simulink model "Completo"  (R2026b)
settings: Solver=ode45  StopTime=10  MaxStep=0.005
libraries: simulink_extras x5
settings Model: Creator=Usuario  LastModifiedBy=Usuario
settings DebuggingCC: UnderSpecifiedDimensionMsg=warning

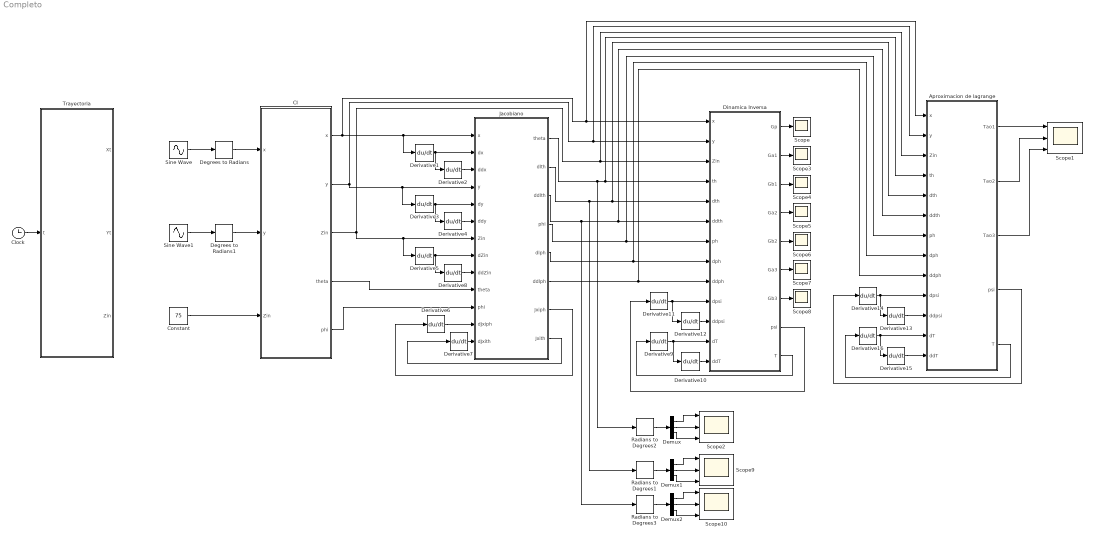
== system Completo ==
  Aproximacion de lagrange : MATLAB Function  TreatAsAtomicUnit=on
  CI : MATLAB Function  TreatAsAtomicUnit=on
  Clock : Clock
  Constant : Constant  Value=75
  Degrees to Radians : simulink_extras/Transformations/Degrees to Radians
  Degrees to Radians1 : simulink_extras/Transformations/Degrees to Radians
  Demux : Demux  Outputs=3
  Demux1 : Demux  Outputs=3
  Demux2 : Demux  Outputs=3
  Derivative{1..16} (16 alike) : Derivative
  Dinamica Inversa : MATLAB Function  TreatAsAtomicUnit=on
  Jacobiano : MATLAB Function  TreatAsAtomicUnit=on
  Radians to Degrees1 : simulink_extras/Transformations/Radians to Degrees
  Radians to Degrees2 : simulink_extras/Transformations/Radians to Degrees
  Radians to Degrees3 : simulink_extras/Transformations/Radians to Degrees
  Scope{,3..8} (7 alike) : Scope
      Scope settings: ActiveDisplayYMinimum=-37.545349688525228  ActiveDisplayYMaximum=37.17658468339345
      Scope3 settings: ActiveDisplayYMinimum=-18.564193111964496  ActiveDisplayYMaximum=37.368196271404251  DataLoggingVariableName=ScopeData3
      Scope4 settings: ActiveDisplayYMinimum=-1  ActiveDisplayYMaximum=1  DataLoggingVariableName=ScopeData4
      Scope5 settings: ActiveDisplayYMinimum=-21.313116337921368  ActiveDisplayYMaximum=32.9435376296142  DataLoggingVariableName=ScopeData5
      Scope6 settings: ActiveDisplayYMinimum=-1  ActiveDisplayYMaximum=1  DataLoggingVariableName=ScopeData6
      Scope7 settings: ActiveDisplayYMinimum=-1  ActiveDisplayYMaximum=1  DataLoggingVariableName=ScopeData7
      Scope8 settings: ActiveDisplayYMinimum=-1  ActiveDisplayYMaximum=1  DataLoggingVariableName=ScopeData8
  Scope{1..2,9..10} (4 alike) : Scope  NumInputPorts=3
      Scope1 settings: ActiveDisplayYMinimum=-0.0048170344652643951  ActiveDisplayYMaximum=-0.0041912233982996754
      Scope10 settings: ActiveDisplayYMinimum=-5322.94377337578  ActiveDisplayYMaximum=5538.32074002052  DataLoggingVariableName=ScopeData10
      Scope2 settings: ActiveDisplayYMinimum=-267.38871393580234  ActiveDisplayYMaximum=-108.53520217148704  DataLoggingVariableName=ScopeData2
      Scope9 settings: ActiveDisplayYMinimum=-34.793520974739913  ActiveDisplayYMaximum=34.948790472185514  DataLoggingVariableName=ScopeData9
  Sine Wave : Sin  Amplitude=10  Frequency=0.5*pi  SampleTime=0
  Sine Wave1 : Sin  Amplitude=10  Frequency=0.5*pi  Phase=pi/2  SampleTime=0
  Trayectoria : MATLAB Function  TreatAsAtomicUnit=on
  wires:
  Derivative6/1 -> Jacobiano/12(dJxiph)
  Derivative7/1 -> Jacobiano/13(dJxith)
  Derivative2/1 -> Jacobiano/3(ddx)
  Derivative1/1 -> Derivative2/1, Jacobiano/2(dx)
  Derivative3/1 -> Jacobiano/5(dy), Derivative4/1
  Derivative4/1 -> Jacobiano/6(ddy)
  Derivative5/1 -> Jacobiano/8(dZin), Derivative8/1
  Derivative8/1 -> Jacobiano/9(ddZin)
  CI/4(theta) -> Jacobiano/10("theta ")
  CI/5(phi) -> Jacobiano/11("phi ")
  Jacobiano/8(Jxith) -> Derivative7/1
  Jacobiano/7(Jxiph) -> Derivative6/1
  Dinamica Inversa/3(Gb1) -> Scope4/1
  Dinamica Inversa/1(Gp) -> Scope/1
  Dinamica Inversa/2(Ga1) -> Scope3/1
  Dinamica Inversa/7(Gb3) -> Scope8/1
  Dinamica Inversa/6(Ga3) -> Scope7/1
  Dinamica Inversa/4(Ga2) -> Scope5/1
  CI/2(y) -> Jacobiano/4(y), Derivative3/1, Dinamica Inversa/2(y), Aproximacion de lagrange/2(y)
  CI/1(x) -> Aproximacion de lagrange/1(x), Dinamica Inversa/1(x), Jacobiano/1(x), Derivative1/1
  Derivative10/1 -> Dinamica Inversa/13(ddT)
  Derivative12/1 -> Dinamica Inversa/11(ddpsi)
  Dinamica Inversa/8(psi) -> Derivative11/1
  Jacobiano/5(dlph) -> Aproximacion de lagrange/8(dph), Dinamica Inversa/8(dph)
  Dinamica Inversa/5(Gb2) -> Scope6/1
  Jacobiano/1(theta) -> Radians to Degrees2/1, Aproximacion de lagrange/4(th), Dinamica Inversa/4(th)
  Jacobiano/6(ddlph) -> Aproximacion de lagrange/9(ddph), Dinamica Inversa/9(ddph)
  Jacobiano/4(phi) -> Aproximacion de lagrange/7(ph), Dinamica Inversa/7(ph)
  Derivative9/1 -> Dinamica Inversa/12(dT), Derivative10/1
  Dinamica Inversa/9(T) -> Derivative9/1
  Derivative11/1 -> Derivative12/1, Dinamica Inversa/10(dpsi)
  Jacobiano/2(dlth) -> Radians to Degrees1/1, Aproximacion de lagrange/5(dth), Dinamica Inversa/5(dth)
  CI/3(Zin) -> Derivative5/1, Jacobiano/7(Zin), Aproximacion de lagrange/3(Zin), Dinamica Inversa/3(Zin)
  Derivative13/1 -> Aproximacion de lagrange/11(ddpsi)
  Derivative14/1 -> Derivative13/1, Aproximacion de lagrange/10(dpsi)
  Derivative15/1 -> Aproximacion de lagrange/13(ddT)
  Derivative16/1 -> Derivative15/1, Aproximacion de lagrange/12(dT)
  Aproximacion de lagrange/5(T) -> Derivative16/1
  Aproximacion de lagrange/4(psi) -> Derivative14/1
  Aproximacion de lagrange/1(Tao1) -> Scope1/1
  Aproximacion de lagrange/2(Tao2) -> Scope1/2
  Aproximacion de lagrange/3(Tao3) -> Scope1/3
  Clock/1 -> Trayectoria/1(t)
  Demux/3 -> Scope2/3
  Demux/1 -> Scope2/1
  Demux/2 -> Scope2/2
  Radians to Degrees2/1 -> Demux/1
  Radians to Degrees1/1 -> Demux1/1
  Demux1/2 -> Scope9/2
  Demux1/1 -> Scope9/1
  Demux1/3 -> Scope9/3
  Demux2/3 -> Scope10/3
  Demux2/1 -> Scope10/1
  Demux2/2 -> Scope10/2
  Radians to Degrees3/1 -> Demux2/1
  Jacobiano/3(ddlth) -> Radians to Degrees3/1, Aproximacion de lagrange/6(ddth), Dinamica Inversa/6(ddth)
  Constant/1 -> CI/3("Zin ")
  Sine Wave/1 -> Degrees to Radians/1
  Degrees to Radians/1 -> CI/1("x ")
  Sine Wave1/1 -> Degrees to Radians1/1
  Degrees to Radians1/1 -> CI/2("y ")

== matlab function Completo/Dinamica Inversa ==
  data: Gp output size=[9,1]; Ga1 output size=[9,1]; Gb1 output size=[9,1]; x input size=[1,1]; Ga2 output size=[9,1]; y input size=[1,1]; Zin input size=[1,1]; Gb2 output size=[9,1]; th input size=[3,1]; dth input size=[3,1]; ddth input size=[3,1]; ph input size=[3,1]; dph input size=[3,1]; ddph input size=[3,1]; dpsi input size=[3,1]; ddpsi input size=[3,1]; dT input size=[3,1]; ddT input size=[3,1]; Ga3 output size=[9,1]; Gb3 output size=[9,1]; psi output size=[3,1]; T output size=[3,1]
function [Gp, Ga1, Gb1, Ga2, Gb2, Ga3, Gb3, psi, T] = fcn(x, y, Zin, th, dth, ddth, ph, dph, ddph, dpsi, ddpsi, dT, ddT)
%% Constantes
p  = 55;
b  = 50;
l1 = 45;
d1 = 19.718;
d2 = 36.703;
dp = 52.00;
%% ============================================================
Ax = x;
Ay = y;
f1 = (-sin(Ax)*sin(Ay))/(cos(Ax)+cos(Ay));
Az = atan(f1);

alfa1 = deg2rad(0);
alfa2 = deg2rad(120);
alfa3 = deg2rad(240);

Oz = Zin;
psi = [Ax; Ay; Az];

R = [cos(Ay)*cos(Az)                        -cos(Ay)*sin(Az)                            sin(Ay)
     cos(Ax)*sin(Az)+cos(Az)*sin(Ax)*sin(Ay) cos(Ax)*cos(Az)-sin(Ax)*sin(Ay)*sin(Az)    -cos(Ay)*sin(Ax)
     sin(Ax)*sin(Az)-cos(Ax)*cos(Az)*sin(Ay) cos(Az)*sin(Ax)+cos(Ax)*sin(Ay)*sin(Az)     cos(Ax)*cos(Ay)];

ux = R(1,1); uy = R(1,2); vy = R(2,2);
Ox = (p*(ux-vy))/2;
Oy = -uy*p;
T  = [Ox; Oy; Oz];

dAx = dpsi(1);
dAy = dpsi(2);
dAz = dpsi(3);

pGp = T + [ dp*sin(Ay)
           -dp*sin(Ax)*cos(Ay)
           -dp*cos(Ax)*cos(Ay)];

JpsiGp = [ 0                    dp*cos(Ay)          0
          -dp*cos(Ax)*cos(Ay)   dp*sin(Ax)*sin(Ay)  0
          -dp*cos(Ay)*sin(Ax)  -dp*cos(Ax)*sin(Ay)  0];

vGp = dT + JpsiGp*dpsi;

dJpsiGp = [ 0                                        -sin(Ay)*dAy                                  0
           (sin(Ax)*cos(Ay)*dAx+cos(Ax)*sin(Ay)*dAy) (cos(Ax)*sin(Ay)*dAx+sin(Ax)*cos(Ay)*dAy)      0
           (sin(Ax)*sin(Ay)*dAy-cos(Ax)*cos(Ay)*dAx) (sin(Ax)*sin(Ay)*dAx-cos(Ax)*cos(Ay)*dAy)      0];

aGp = ddT + dJpsiGp*dpsi + JpsiGp*ddpsi;

Gp = [pGp; vGp; aGp];

[pGth1, vGth1, aGth1, pGph1, vGph1, aGph1] = solve(th(1), dth(1), ddth(1), ph(1), dph(1), ddph(1), alfa1, b, l1, d1, d2);
[pGth2, vGth2, aGth2, pGph2, vGph2, aGph2] = solve(th(2), dth(2), ddth(2), ph(2), dph(2), ddph(2), alfa2, b, l1, d1, d2);
[pGth3, vGth3, aGth3, pGph3, vGph3, aGph3] = solve(th(3), dth(3), ddth(3), ph(3), dph(3), ddph(3), alfa3, b, l1, d1, d2);

Ga1 = [pGth1; vGth1; aGth1];
Gb1 = [pGph1; vGph1; aGph1];
Ga2 = [pGth2; vGth2; aGth2];
Gb2 = [pGph2; vGph2; aGph2];
Ga3 = [pGth3; vGth3; aGth3];
Gb3 = [pGph3; vGph3; aGph3];

end % <-- cierre de fcn (ver nota abajo)


function [pGi, vGi, aGi, pGj, vGj, aGj] = solve(theta_i, dth_i, ddth_i, phi_i, dphi_i, ddphi_i, alfa_i, b, l1, d1, d2)

pGi = [cos(alfa_i)*(b + d1*cos(theta_i));
       sin(alfa_i)*(b + d1*cos(theta_i));
       -d1*sin(theta_i)];

JthGi = -[d1*cos(alfa_i)*sin(theta_i);
          d1*sin(alfa_i)*sin(theta_i);
          d1*cos(theta_i)];

vGi = JthGi*dth_i;

dJthGi = [-d1*cos(alfa_i)*cos(theta_i);
          -d1*sin(alfa_i)*cos(theta_i);
           d1*sin(theta_i)];

aGi = dJthGi*dth_i + JthGi*ddth_i;

pGj = [cos(alfa_i)*(b + l1*cos(theta_i) + d2*cos(phi_i));
       sin(alfa_i)*(b + l1*cos(theta_i) + d2*cos(phi_i));
       -l1*sin(theta_i) - d2*sin(phi_i)];

JthGj = -[l1*cos(alfa_i)*sin(theta_i);
          l1*sin(alfa_i)*sin(theta_i);
          l1*cos(theta_i)];

JphGj = -[d2*cos(alfa_i)*sin(phi_i);
          d2*sin(alfa_i)*sin(phi_i);
          d2*cos(phi_i)];

vGj = JthGj*dth_i + JphGj*dphi_i;

dJthGj = [-l1*cos(alfa_i)*cos(theta_i);
          -l1*sin(alfa_i)*cos(theta_i);
           l1*sin(theta_i)];

dJphGj = [-d2*cos(alfa_i)*cos(phi_i);
          -d2*sin(alfa_i)*cos(phi_i);
           d2*sin(phi_i)];

aGj = dJthGj*dth_i + JthGj*ddth_i + dJphGj*dphi_i + JphGj*ddphi_i;

end

== matlab function Completo/CI ==
  data: x output; y output; Zin output; x input; theta output; y input; Zin input; phi output
function [x,y,Zin,theta, phi] = fcn(x,y, Zin)
%%constantes
p  = 55;   
b  = 50;    
l1 = 45;   
l2 = 75;  
%% ============================================================
Ax = x;
Ay = y;
f1=(-sin(Ax)*sin(Ay))/(cos(Ax)+cos(Ay));
Az=atan(f1);
alfa1 = deg2rad(0);
alfa2 = deg2rad(120);
alfa3 = deg2rad(240);
Oz = Zin;

R = [ cos(Ay)*cos(Az)                          -cos(Ay)*sin(Az)                          sin(Ay)
      cos(Ax)*sin(Az)+cos(Az)*sin(Ax)*sin(Ay)    cos(Ax)*cos(Az)-sin(Ax)*sin(Ay)*sin(Az)  -cos(Ay)*sin(Ax)
      sin(Ax)*sin(Az)-cos(Ax)*cos(Az)*sin(Ay)    cos(Az)*sin(Ax)+cos(Ax)*sin(Ay)*sin(Az)   cos(Ax)*cos(Ay)];
Rz1 = [cos(alfa1) -sin(alfa1) 0; sin(alfa1) cos(alfa1) 0; 0 0 1];
Rz2 = [cos(alfa2) -sin(alfa2) 0; sin(alfa2) cos(alfa2) 0; 0 0 1];
Rz3 = [cos(alfa3) -sin(alfa3) 0; sin(alfa3) cos(alfa3) 0; 0 0 1];
P = [p; 0; 0];
ux = R(1,1); uy = R(1,2); vy = R(2,2);
Ox = (p*(ux-vy))/2;
Oy = -uy*p;
T  = [Ox, Oy, Oz];
O1 = T' + (R*Rz1*P);
O2 = T' + (R*Rz2*P);
O3 = T' + (R*Rz3*P);

%% ============================================================
    function [th,phi] = solveLeg(O, alfa, b, l1, l2)
    A = 2*l1*cos(alfa)*(b*cos(alfa) - O(1));
    B = 2*l1*O(3)*cos(alfa)^2;
    C = O(1)^2 - 2*b*O(1)*cos(alfa) + cos(alfa)^2*(b^2 + l1^2 - l2^2 + O(3)^2);

    %disc = A^2 + B^2 - C^2;   % si es negativo -> pose inalcanzable
    f_sol1 =(+B+sqrt(A^2+B^2-C^2))\(C-A);
    % f_sol2 = (C - A) / (-B - sqrt(disc)); 

    Ang1 = 2*atan(f_sol1);
    th = (-Ang1)-pi; 

    Cphi11=(O(1)-cos(alfa)*(b+l1*cos(th)))/(l2*cos(alfa));
    Sphi11=(-O(3)+l1*sin(th))/l2;

    phi=(atan2(Cphi11,Sphi11))+pi/2;
    end
[theta1,phi1] = solveLeg(O1, alfa1, b, l1, l2);
[theta2,phi2] = solveLeg(O2, alfa2, b, l1, l2);
[theta3,phi3] = solveLeg(O3, alfa3, b, l1, l2);

theta=[theta1;theta2;theta3];
phi=[phi1;phi2;phi3];
end

== matlab function Completo/Aproximacion de lagrange ==
  data: Tao1 output size=[1,1]; Tao2 output size=[1,1]; Tao3 output size=[1,1]; x input size=[1,1]; y input size=[1,1]; Zin input size=[1,1]; th input size=[3,1]; dth input size=[3,1]; ddth input size=[3,1]; ph input size=[3,1]; dph input size=[3,1]; ddph input size=[3,1]; dpsi input size=[3,1]; ddpsi input size=[3,1]; dT input size=[3,1]; ddT input size=[3,1]; psi output size=[3,1]; T output size=[3,1]
function [Tao1, Tao2, Tao3, psi,T] = fcn(x, y, Zin, th, dth, ddth, ph, dph, ddph, dpsi, ddpsi, dT,ddT)
%%constantes
p  = 55; %mm   
b  = 50;    
l1 = 45;   
l2 = 75;  
d1 = 19.718; 
d2 = 36.703;
dp = 52.00;
m1 = 3.18; %gramos
m2 = 4.36;
mp = 43.32;
I1yy = 652.49;
I2yy = 519.69;
IPx = 21311.68;
IPy = 42281.84;
IPz = 21311.66;
g = 9810; %mm/s2
%% ============================================================
Ax = x;
Ay = y;
f1=(-sin(Ax)*sin(Ay))/(cos(Ax)+cos(Ay));
Az=atan(f1);

alfa1 = deg2rad(0);
alfa2 = deg2rad(120);
alfa3 = deg2rad(240);
R = [ cos(Ay)*cos(Az)                          -cos(Ay)*sin(Az)                          sin(Ay)
    cos(Ax)*sin(Az)+cos(Az)*sin(Ax)*sin(Ay)    cos(Ax)*cos(Az)-sin(Ax)*sin(Ay)*sin(Az)  -cos(Ay)*sin(Ax)
    sin(Ax)*sin(Az)-cos(Ax)*cos(Az)*sin(Ay)    cos(Az)*sin(Ax)+cos(Ax)*sin(Ay)*sin(Az)   cos(Ax)*cos(Ay)];
ux = R(1,1); uy = R(1,2); vy = R(2,2);
Ox = (p*(ux-vy))/2;
Oy = -uy*p;
Oz = Zin;
T = [Ox;Oy;Oz];
psi = [Ax; Ay; Az];
psix=Ax; psiy=Ay; psiz=Az; 

th1 = th(1); th2 = th(2); th3 = th(3);
dth1 = dth(1); dth2 = dth(2); dth3 = dth(3);
ddth1 = ddth(1); ddth2 = ddth(2); ddth3 = ddth(3);
ph1 = ph(1); ph2 = ph(2); ph3 = ph(3);
dph1 = dph(1); dph2 = dph(2); dph3 = dph(3);
ddph1 = ddph(1); ddph2 = ddph(2); ddph3 = ddph(3);
dpsix = dpsi(1); dpsiy = dpsi(2); dpsiz = dpsi(3);
ddpsix = ddpsi(1); ddpsiy = ddpsi(2); ddpsiz = ddpsi(3);
dOx = dT(1); dOy = dT(2); dOz = dT(3);
ddOx = ddT(1); ddOy = ddT(2); ddOz = ddT(3);
%% lagrangiano
L1 = g*(-d1*m1 - l2*m2)*cos(th1) + d2*l2*m2*sin(th1 - ph1)*dph1^2+ (I1yy + d1^2*m1 + l2^2*m2)*ddth1 + d2*l2*m2*cos(th1 - ph1)*ddph1;
L2 = g*(-d1*m1 - l2*m2)*cos(th2) + d2*l2*m2*sin(th2 - ph2)*dph2^2+ (I1yy + d1^2*m1 + l2^2*m2)*ddth2 + d2*l2*m2*cos(th2 - ph2)*ddph2;
L3 = g*(-d1*m1 - l2*m2)*cos(th3) + d2*l2*m2*sin(th3 - ph3)*dph3^2+ (I1yy + d1^2*m1 + l2^2*m2)*ddth3 + d2*l2*m2*cos(th3 - ph3)*ddph3;
L4 = -d2*g*m2*cos(ph1) + I2yy*ddph1 + d2*m2*(-l2*sin(th1 - ph1)*dth1^2 + l2*cos(th1 - ph1)*ddth1 + d2*ddph1);
L5 = -d2*g*m2*cos(ph2) + I2yy*ddph2 + d2*m2*(-l2*sin(th2 - ph2)*dth2^2 + l2*cos(th2 - ph2)*ddth2 + d2*ddph2);
L6 = -d2*g*m2*cos(ph3) + I2yy*ddph3 + d2*m2*(-l2*sin(th3 - ph3)*dth3^2 + l2*cos(th3 - ph3)*ddth3 + d2*ddph3);
L7 = mp*(-dp*sin(psiy)*dpsiy^2 + ddOx + dp*cos(psiy)*ddpsiy);
L8 = mp*(ddOy + dp*(sin(psix)*cos(psiy)*dpsix^2 + 2*cos(psix)*sin(psiy)*dpsix*dpsiy + sin(psix)*cos(psiy)*dpsiy^2 - cos(psix)*cos(psiy)*ddpsix + sin(psix)*sin(psiy)*ddpsiy));
L9 = mp*(g + ddOz + dp*(- cos(psix)*cos(psiy)*dpsix^2 + 2*sin(psix)*sin(psiy)*dpsix*dpsiy + cos(psix)*cos(psiy)*dpsiy^2 - sin(psix)*cos(psiy)*ddpsix - cos(psix)*sin(psiy)*ddpsiy));
L10 = -dp*g*mp*sin(psix)*cos(psiy) - dp^2*mp*sin(2*psiy)*dpsix*dpsiy + 0.5*(IPy - IPz)*sin(2*psix)*dpsiy^2 - dp*mp*cos(psix)*cos(psiy)*ddOy + (IPx + (IPy - IPz)*cos(2*psix))*cos(psiy)*dpsiy*dpsiz - IPy*cos(psix)*sin(psix)*cos(psiy)^2*dpsiz^2 + 0.5*IPz*sin(2*psix)*cos(psiy)^2*dpsiz^2 - dp*mp*sin(psix)*cos(psiy)*ddOz + IPx*ddpsix + 0.5*dp^2*mp*ddpsix + 0.5*dp^2*mp*cos(2*psiy)*ddpsix + IPx*sin(psiy)*ddpsiz;
L11 = -dp*g*mp*cos(psix)*sin(psiy) + 0.5*dp^2*mp*sin(2*psiy)*dpsix^2 + 0.5*(IPz*cos(psix)^2*sin(2*psiy) + (-IPx + IPy*sin(psix)^2)*sin(2*psiy) )*dpsiz^2 + dpsix*(-IPx*cos(psiy)*dpsiz + (-IPy + IPz)*(sin(2*psix)*dpsiy + cos(2*psix)*cos(psiy)*dpsiz)) + dp*mp*cos(psiy)*ddOx + dp*mp*sin(psix)*sin(psiy)*ddOy - dp*mp*cos(psix)*sin(psiy)*ddOz + 0.5*(IPy + IPz)*ddpsiy + dp^2*mp*ddpsiy + 0.5*cos(2*psix)*(IPy - IPz)*ddpsiy - 0.5*sin(2*psix)*cos(psiy)*(IPy - IPz)*ddpsiz;
L12 = 0.5*(IPy - IPz)*sin(2*psix)*sin(psiy)*dpsiy^2 + (-IPz*cos(psix)^2 + (IPx - IPy*sin(psix)^2))*sin(2*psiy)*dpsiy*dpsiz + (IPx + (-IPy + IPz)*cos(2*psix))*cos(psiy)*dpsix*dpsiy + (IPy - IPz)*sin(2*psix)*cos(psiy)^2*dpsix*dpsiz + (0.5*(-IPy + IPz)*sin(2*psix)*cos(psiy)*ddpsiy + (IPz*cos(psix)^2 + IPy*sin(psix)^2)*cos(psiy)^2*ddpsiz) + IPx*sin(psiy)*(ddpsix + sin(psiy)*ddpsiz);

Lagrange1=[L1;L2;L3];
Lagrange2=[L4;L5;L6;L7;L8;L9;L10;L11;L12]; %Fuerzas externas sobre L7, L8, L9 (x,y,z)
%% matriz gamma
Gamma1 = ...
[-l1*cos(alfa1)*sin(th1), -l1*sin(alfa1)*sin(th1), l1*cos(th1),                                                                                 0,                                                                                 0,                                             0,                                                                                 0,                                                                                 0,                                               0
                       0,                       0,           0,                                                           -l1*cos(alfa2)*sin(th2),                                                           -l1*sin(alfa2)*sin(th2),                                   l1*cos(th2),                                                                                 0,                                                                                 0,                                               0
                       0,                       0,           0,                                                                                 0,                                                                                 0,                                             0,                                                           -l1*cos(alfa3)*sin(th3),                                                           -l1*sin(alfa3)*sin(th3),                                     l1*cos(th3)];
Gamma2 = ...
[-l2*cos(alfa1)*sin(ph1), -l2*sin(alfa1)*sin(ph1), l2*cos(ph1),                                                                                 0,                                                                                 0,                                             0,                                                                                 0,                                                                                 0,                                               0
                       0,                       0,           0,                                                           -l2*cos(alfa2)*sin(ph2),                                                           -l2*sin(alfa2)*sin(ph2),                                   l2*cos(ph2),                                                                                 0,                                                                                 0,                                               0
                       0,                       0,           0,                                                                                 0,                                                                                 0,                                             0,                                                           -l2*cos(alfa3)*sin(ph3),                                                           -l2*sin(alfa3)*sin(ph3),                                     l2*cos(ph3)
                       1,                       0,           0,                                                                                 1,                                                                                 0,                                             0,                                                                                 1,                                                                                 0,                                               0
                       0,                       1,           0,                                                                                 0,                                                                                 1,                                             0,                                                                                 0,                                                                                 1,                                               0
                       0,                       0,           1,                                                                                 0,                                                                                 0,                                             1,                                                                                 0,                                                                                 0,                                               1
                       0,                       0,           0,                        -(3^(1/2)*p*(sin(Ax)*sin(Az) - cos(Ax)*cos(Az)*sin(Ay)))/2,                        -(3^(1/2)*p*(cos(Az)*sin(Ax) + cos(Ax)*sin(Ay)*sin(Az)))/2,                -(3^(1/2)*p*cos(Ax)*cos(Ay))/2,                         (3^(1/2)*p*(sin(Ax)*sin(Az) - cos(Ax)*cos(Az)*sin(Ay)))/2,                         (3^(1/2)*p*(cos(Az)*sin(Ax) + cos(Ax)*sin(Ay)*sin(Az)))/2,                   (3^(1/2)*p*cos(Ax)*cos(Ay))/2
      -p*cos(Az)*sin(Ay),       p*sin(Ay)*sin(Az),   p*cos(Ay),                     (p*cos(Az)*sin(Ay))/2 + (3^(1/2)*p*cos(Ay)*cos(Az)*sin(Ax))/2,                   - (p*sin(Ay)*sin(Az))/2 - (3^(1/2)*p*cos(Ay)*sin(Ax)*sin(Az))/2, (3^(1/2)*p*sin(Ax)*sin(Ay))/2 - (p*cos(Ay))/2,                     (p*cos(Az)*sin(Ay))/2 - (3^(1/2)*p*cos(Ay)*cos(Az)*sin(Ax))/2,                     (3^(1/2)*p*cos(Ay)*sin(Ax)*sin(Az))/2 - (p*sin(Ay)*sin(Az))/2, - (p*cos(Ay))/2 - (3^(1/2)*p*sin(Ax)*sin(Ay))/2
      -p*cos(Ay)*sin(Az),      -p*cos(Ay)*cos(Az),           0, (p*cos(Ay)*sin(Az))/2 + (3^(1/2)*p*(cos(Ax)*cos(Az) - sin(Ax)*sin(Ay)*sin(Az)))/2, (p*cos(Ay)*cos(Az))/2 - (3^(1/2)*p*(cos(Ax)*sin(Az) + cos(Az)*sin(Ax)*sin(Ay)))/2,                                             0, (p*cos(Ay)*sin(Az))/2 - (3^(1/2)*p*(cos(Ax)*cos(Az) - sin(Ax)*sin(Ay)*sin(Az)))/2, (p*cos(Ay)*cos(Az))/2 + (3^(1/2)*p*(cos(Ax)*sin(Az) + cos(Az)*sin(Ax)*sin(Ay)))/2,                                               0];

%% Matriz lambda y torques
Lambda= (inv(Gamma2))*Lagrange2;
Ta= Lagrange1 + Gamma1*Lambda;
Tao= Ta*10^-9;
Tao1=Tao(1); Tao2=Tao(2); Tao3=Tao(3);
end

== matlab function Completo/Jacobiano ==
  data: theta output; x input; dx input; ddx input; dlth output; ddlth output; phi output; y input; dy input; ddy input; Zin input; dZin input; ddZin input; dlph output; ddlph output; theta input; phi input; dJxiph input; Jxiph output; Jxith output; dJxith input
function [theta,dlth,ddlth,phi, dlph,ddlph, Jxiph, Jxith] = fcn(x,dx,ddx,y,dy,ddy,Zin,dZin,ddZin,theta, phi,dJxiph,dJxith)
%% Constantes
p  = 55;
b  = 50;
l1 = 45;
l2 = 75;
Ax = x;
Ay = y;
f1 = (-sin(Ax)*sin(Ay))/(cos(Ax)+cos(Ay));
Az = atan(f1);
alfa1 = deg2rad(0);
alfa2 = deg2rad(120);
alfa3 = deg2rad(240);
Oz = Zin;

R = [ cos(Ay)*cos(Az)                          -cos(Ay)*sin(Az)                          sin(Ay)
      cos(Ax)*sin(Az)+cos(Az)*sin(Ax)*sin(Ay)    cos(Ax)*cos(Az)-sin(Ax)*sin(Ay)*sin(Az)  -cos(Ay)*sin(Ax)
      sin(Ax)*sin(Az)-cos(Ax)*cos(Az)*sin(Ay)    cos(Az)*sin(Ax)+cos(Ax)*sin(Ay)*sin(Az)   cos(Ax)*cos(Ay)];

Rz1 = [cos(alfa1) -sin(alfa1) 0; sin(alfa1) cos(alfa1) 0; 0 0 1];
Rz2 = [cos(alfa2) -sin(alfa2) 0; sin(alfa2) cos(alfa2) 0; 0 0 1];
Rz3 = [cos(alfa3) -sin(alfa3) 0; sin(alfa3) cos(alfa3) 0; 0 0 1];

P = [p; 0; 0];
ux = R(1,1); 
uy = R(1,2); 
vy = R(2,2);
Ox = (p*(ux-vy))/2;
Oy = -uy*p;
T  = [Ox; Oy; Oz];
O1 = T + (R*Rz1*P); O2 = T + (R*Rz2*P); O3 = T + (R*Rz3*P);

th1 = theta(1); th2 = theta(2); th3 = theta(3);
phi1 = phi(1); phi2 = phi(2); phi3 = phi(3);
%% Jacobiano de la restricción de cada pierna (lD, E)
lD1 = [-2*cos(alfa1)*(b+l1*cos(th1))+2*O1(1)   0   2*cos(alfa1)^2*(O1(3)+l1*sin(th1))];
E1  =  2*l1*cos(alfa1)*(cos(alfa1)*cos(th1)*O1(3) + (-b*cos(alfa1)+O1(1))*sin(th1));

lD2 = [-2*cos(alfa2)*(b+l1*cos(th2))+2*O2(1)   0   2*cos(alfa2)^2*(O2(3)+l1*sin(th2))];
E2  =  2*l1*cos(alfa2)*(cos(alfa2)*cos(th2)*O2(3) + (-b*cos(alfa2)+O2(1))*sin(th2));

lD3 = [-2*cos(alfa3)*(b+l1*cos(th3))+2*O3(1)   0   2*cos(alfa3)^2*(O3(3)+l1*sin(th3))];
E3  =  2*l1*cos(alfa3)*(cos(alfa3)*cos(th3)*O3(3) + (-b*cos(alfa3)+O3(1))*sin(th3));

Js = [lD1  0  0  0  0  0  0
       0   0  0 lD2 0  0  0
       0   0  0  0  0  0 lD3];

Jth = [E1  0  0
        0  E2 0
        0  0  E3];
dlX=[dZin; dx; dy];

%% Jacobiano de orientación pierna<-plataforma 
Jto1 = [1 0 0                    0                                           (-p*sin(Ay)*cos(alfa1+Az))              (-p*cos(Ay)*sin(alfa1+Az))
        0 1 0 p*((cos(Ax)*sin(Ay)*cos(alfa1+Az))-sin(Ax)*sin(alfa1+Az))  (p*sin(Ax)*cos(Ay)*cos(alfa1+Az))  p*(cos(Ax)*cos(alfa1+Az)-(sin(Ax)*sin(Ay)*sin(alfa1+Az)))
        0 0 1 p*((sin(Ax)*sin(Ay)*cos(alfa1+Az))+cos(Ax)*sin(alfa1+Az)) (-p*cos(Ax)*cos(Ay)*cos(alfa1+Az))  p*(sin(Ax)*cos(alfa1+Az)+(cos(Ax)*sin(Ay)*sin(alfa1+Az)))];

Jto2 = [1 0 0                    0                                           (-p*sin(Ay)*cos(alfa2+Az))              (-p*cos(Ay)*sin(alfa2+Az))
        0 1 0 p*((cos(Ax)*sin(Ay)*cos(alfa2+Az))-sin(Ax)*sin(alfa2+Az))  (p*sin(Ax)*cos(Ay)*cos(alfa2+Az))  p*(cos(Ax)*cos(alfa2+Az)-(sin(Ax)*sin(Ay)*sin(alfa2+Az)))
        0 0 1 p*((sin(Ax)*sin(Ay)*cos(alfa2+Az))+cos(Ax)*sin(alfa2+Az)) (-p*cos(Ax)*cos(Ay)*cos(alfa2+Az))  p*(sin(Ax)*cos(alfa2+Az)+(cos(Ax)*sin(Ay)*sin(alfa2+Az)))];

Jto3 = [1 0 0                    0                                           (-p*sin(Ay)*cos(alfa3+Az))              (-p*cos(Ay)*sin(alfa3+Az))
        0 1 0 p*((cos(Ax)*sin(Ay)*cos(alfa3+Az))-sin(Ax)*sin(alfa3+Az))  (p*sin(Ax)*cos(Ay)*cos(alfa3+Az))  p*(cos(Ax)*cos(alfa3+Az)-(sin(Ax)*sin(Ay)*sin(alfa3+Az)))
        0 0 1 p*((sin(Ax)*sin(Ay)*cos(alfa3+Az))+cos(Ax)*sin(alfa3+Az)) (-p*cos(Ax)*cos(Ay)*cos(alfa3+Az))  p*(sin(Ax)*cos(alfa3+Az)+(cos(Ax)*sin(Ay)*sin(alfa3+Az)))];

Jts = [Jto1; Jto2; Jto3];

%% Jacobiano de la tarea independiente 
Jox = [0 -(p*cos(Ay)*sin(Ay)*(cos(Ax)+cos(Ay)*sin(Ax)*sin(Ay)))/(2*(1+cos(Ax)*cos(Ay))^2) ...
         -(p*cos(Ay)*sin(Ax)*(cos(Ax)+cos(Ay)+sin(Ax)*sin(Ay)))/(2*(1+cos(Ax)*cos(Ay))^2)];
Joy = [0 -(p*cos(Ay)*sin(Ay)*(cos(Ax)+cos(Ay)))/((1+cos(Ax)*cos(Ay))^2) ...
         -(p*sin(Ax)*(sin(Ax)^2*sin(Ay)^2-cos(Ay)^4-cos(Ax)^2*cos(Ay)^2-1/4*cos(Ax)*(5*cos(Ay)+3*cos(Ay)^3)))/((1+cos(Ax)*cos(Ay))^3)];
JAz = [0 -sin(Ay)/(1+cos(Ax)*cos(Ay))  -sin(Ax)/(1+cos(Ax)*cos(Ay))];
I3x3 = eye(3);

Jxit = [Jox; Joy; I3x3; JAz];
Jxith = (-inv(Jth))*Js*Jts*Jxit; 
Dlth=Jxith*dlX;
dlth=[Dlth(1);Dlth(2);Dlth(3)]

JSph1 = [0 0 -1/l2*cos(phi1)];
Jth1ph1 = -l1*cos(th1)/l2*cos(phi1);
JSph2 = [0 0 -1/l2*cos(phi2)];
Jth2ph2 = -l1*cos(th2)/l2*cos(phi2);
JSph3 = [0 0 -1/l2*cos(phi3)];
Jth3ph3 = -l1*cos(th3)/l2*cos(phi3);

JSph = [JSph1 0 0   0   0 0   0
          0   0 0 JSph2 0 0   0
          0   0 0   0   0 0 JSph3];
Jthph = [Jth1ph1    0        0
            0    Jth2ph2     0
            0       0    Jth3ph3];

Jxis  = Jts*Jxit;
Jxiph = (JSph*Jxis + Jthph*Jxith);   
Dlph=Jxiph*dlX;
dlph=[Dlph(1);Dlph(2);Dlph(3)];
%%segunda derivada
ddlX=[ddZin;ddx;ddy];
Ddlth=dJxith*dlX+Jxith*ddlX;
ddlth=[Ddlth(1);Ddlth(2);Ddlth(3)]
Ddlph=dJxiph*dlX+Jxiph*ddlX;
ddlph=[Ddlph(1);Ddlph(2);Ddlph(3)];
end

== matlab function Completo/Trayectoria ==
  data: Xt output; Yt output; Zin output; t input
function [Xt, Yt, Zin] = fcn(t)

w   = 0.5*pi;    % frecuencia angular del seno en X,Y [rad/s]
amp = 10;      % amplitud de X,Y

t1 = 5;        % fin rampa de subida (60 -> 75)
t2 = 15;       % fin de la fase senoidal (10 s)
t3 = 20;       % fin rampa de bajada (75 -> 60)

tRise = 0.5;   % duración del fundido de entrada/salida de la amplitud [s]

if t < t1
    % Rampa de subida: Z va de 60 a 75 en 5 s
    Zin = 60 + 15*(t/t1);
    Xt  = 0;
    Yt  = 0;

elseif t < t2
    % Z estable en 75, X,Y en seno con envolvente suave (sin saltos)
    Zin = 75;
    tau = t - t1;                                   % tiempo dentro de la fase (0..10)

    % envolvente: sube en [0, tRise], baja en [10-tRise, 10]
    envIn  = min(1, tau/tRise);
    envOut = min(1, (t2 - t1 - tau)/tRise);
    env    = min(envIn, envOut);

    Xt = amp*env*cos(w*tau);
    Yt = amp*env*sin(w*tau);

elseif t < t3
    % Rampa de bajada: Z vuelve de 75 a 60 en 5 s, X,Y ya en 0 (sin salto)
    Zin = 75 - 15*((t - t2)/(t3 - t2));
    Xt  = 0;
    Yt  = 0;

else
    % Reposo final en el punto inicial
    Zin = 60;
    Xt  = 0;
    Yt  = 0;
end
